simulink model "hydro_physics"  (R2026a)
settings: Solver=VariableStepAuto
settings Model: Creator=hrish  LastModifiedBy=hrish
settings DataIOCC: ExternalInput=sim_input  LoadExternalInput=on

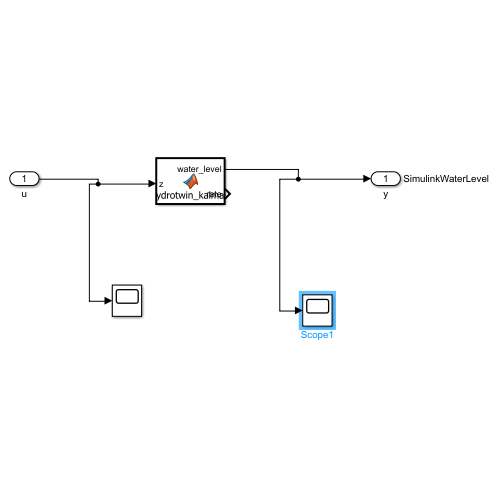
[thumbnail: Simulink's stored preview of the top-level diagram]
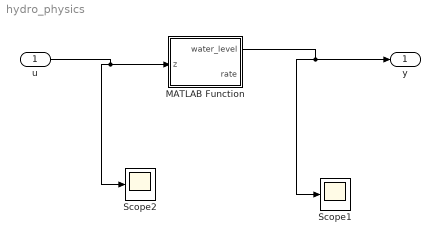
== system hydro_physics ==
  u : Inport
  MATLAB Function : MATLAB Function  TreatAsAtomicUnit=on
  Scope1 : Scope
      settings: ActiveDisplayYMinimum=-1  ActiveDisplayYMaximum=1
  Scope2 : Scope
      settings: ActiveDisplayYMinimum=-1  ActiveDisplayYMaximum=1
  y : Outport  SignalName=SimulinkWaterLevel
  wires:
  MATLAB Function/1(water_level) -> y/1, Scope1/1
  u/1 -> MATLAB Function/1(z), Scope2/1

== matlab function hydro_physics/MATLAB Function ==
  data: z input; water_level output; rate output
function [water_level, rate] = hydrotwin_kalman(z)
%#codegen
% Exact Kalman + sensor-health logic used in HydroTwin main code

persistent x_est P previous_z first_sample

if isempty(x_est)
    % Initial Kalman state
    x_est = [1.0;
             0.0];

    % Initial covariance
    P = [1 0;
         0 1];

    previous_z = 0;
    first_sample = true;
end

% ========================================================================
% CONSTANTS — SAME AS MAIN MATLAB CODE
% ========================================================================

dt = 1;

F = [1 dt;
     0 0.96];

H = [1 0];

Q = [0.015 0;
     0     0.010];

R = 0.20^2;

% ========================================================================
% STEP 1 — SENSOR HEALTH
% ========================================================================

% ML anomaly detection is disabled in the current main:
% use_ml_model = false

ml_anomaly = false;

% Physical sensor failure
physical_failure = ...
    (z < 0.20) || ...
    (z > 12.0);

% Rate-based failure detection
if first_sample
    unrealistic_rate = false;
    first_sample = false;
else
    rate_measurement = (z - previous_z) / dt;

    unrealistic_rate = ...
        abs(rate_measurement) > 1.5;
end

% Overall sensor health
sensor_broken = ...
    ml_anomaly || ...
    physical_failure || ...
    unrealistic_rate;

% Store current sensor value for next sample
previous_z = z;

% ========================================================================
% STEP 2 — KALMAN PREDICTION
% ========================================================================

x_pred = F * x_est;

P_pred = F * P * F' + Q;

% ========================================================================
% STEP 3 — SENSOR FUSION / FAILSAFE
% ========================================================================

if sensor_broken

    % Sensor failed:
    % MODEL-ONLY PREDICTION
    x_est = x_pred;
    P = P_pred;

else

    % Sensor healthy:
    % NORMAL KALMAN MEASUREMENT UPDATE

    innovation = z - H * x_pred;

    innovation_cov = ...
        H * P_pred * H' + R;

    K = P_pred * H' / innovation_cov;

    x_est = ...
        x_pred + K * innovation;

    P = ...
        (eye(2) - K * H) * P_pred;
end

% ========================================================================
% STEP 4 — PHYSICAL LIMITS
% ========================================================================

x_est(1) = max(x_est(1), 0);

x_est(2) = ...
    max(min(x_est(2), 2), -2);

% ========================================================================
% OUTPUTS
% ========================================================================

water_level = x_est(1);

rate = x_est(2);
